simulink model "chap14t1"  (R2022b)
settings: Solver=VariableStepAuto  StartTime=0.0  StopTime=10.0  RelTol=1e-3
libraries: simulink x1
settings Model: Creator=hp  LastModifiedBy=hp

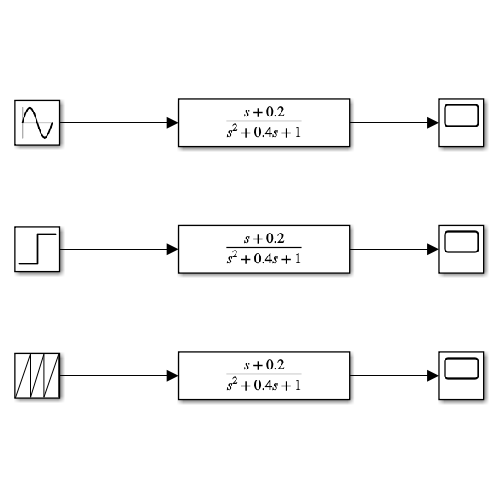
[thumbnail: Simulink's stored preview of the top-level diagram]
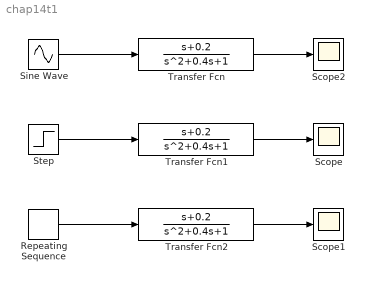
== system chap14t1 ==
  Repeating Sequence : simulink/Sources/Repeating Sequence  rep_seq_t=[0 2]  rep_seq_y=[0 2]
  Scope : Scope
  Scope1 : Scope
  Scope2 : Scope
  Sine Wave : Sin  SampleTime=0
  Step : Step  SampleTime=0
  Transfer Fcn : TransferFcn  Numerator=[1 0.2]  Denominator=[1 0.4 1]
  Transfer Fcn1 : TransferFcn  Numerator=[1 0.2]  Denominator=[1 0.4 1]
  Transfer Fcn2 : TransferFcn  Numerator=[1 0.2]  Denominator=[1 0.4 1]
  wires:
  Sine Wave/1 -> Transfer Fcn/1
  Step/1 -> Transfer Fcn1/1
  Repeating Sequence/1 -> Transfer Fcn2/1
  Transfer Fcn1/1 -> Scope/1
  Transfer Fcn2/1 -> Scope1/1
  Transfer Fcn/1 -> Scope2/1
